simulink model "Gr3_Ex1_3linkedRobot_old"  (R2024b)
settings: Solver=VariableStepAuto  StartTime=0.0  StopTime=10.0  RelTol=1e-3
settings Model: Creator=UX434  LastModifiedBy=UX434

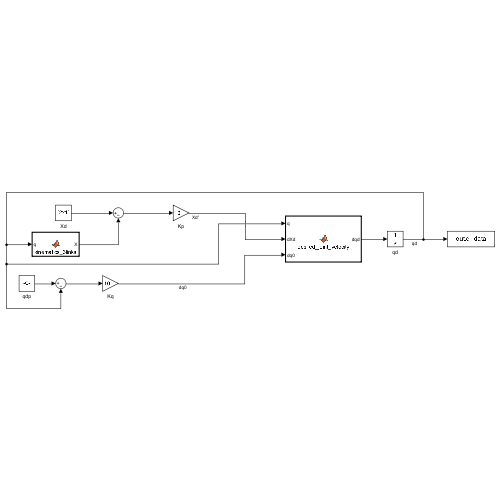
[thumbnail: Simulink's stored preview of the top-level diagram]
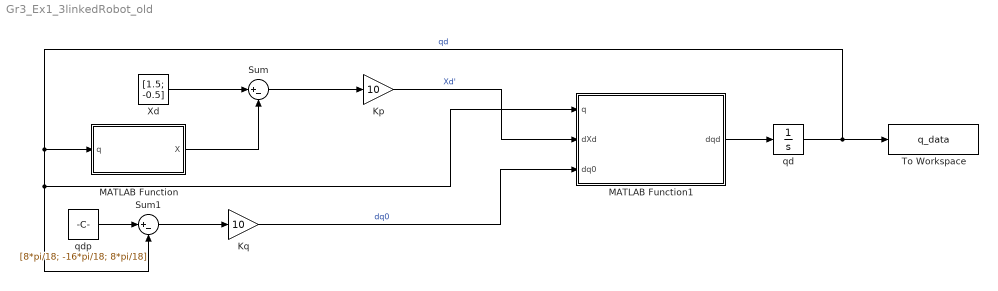
== system Gr3_Ex1_3linkedRobot_old ==
  Kp : Gain  Gain=10
  Kq : Gain  Gain=10
  MATLAB Function : MATLAB Function  TreatAsAtomicUnit=on
  MATLAB Function1 : MATLAB Function  TreatAsAtomicUnit=on
  Sum : Sum  Inputs=|+-
  Sum1 : Sum  Inputs=|+-
  To Workspace : ToWorkspace  VariableName=q_data  SampleTime=-1
  Xd : Constant  Value=[1.5; -0.5]
  qd : Integrator  InitialCondition=[pi/12; pi/3; pi/3]
  qdp : Constant  Value=[8*pi/18; -16*pi/18; 8*pi/18]
  wires:
  qd/1 -> To Workspace/1, MATLAB Function1/1(q), Sum1/2, MATLAB Function/1(q)  "qd"
  MATLAB Function/1(X) -> Sum/2
  Sum/1 -> Kp/1
  Kp/1 -> MATLAB Function1/2(dXd)  "Xd'"
  qdp/1 -> Sum1/1
  Sum1/1 -> Kq/1
  Kq/1 -> MATLAB Function1/3(dq0)  "dq0"
  MATLAB Function1/1(dqd) -> qd/1
  Xd/1 -> Sum/1

== matlab function Gr3_Ex1_3linkedRobot_old/MATLAB Function ==
  data: q input; X output
function X = kinematics_3links(q)
    l1 = 1;  l2 = 1;  l3 = 0.3;
    s1 = sin(q(1));  s12 = sin(q(1)+q(2));  s123 = sin(q(1)+q(2)+q(3));
    c1 = cos(q(1));  c12 = cos(q(1)+q(2));  c123 = cos(q(1)+q(2)+q(3));
    X = [l1*c1 + l2*c12 + l3*c123;
         l1*s1 + l2*s12 + l3*s123];
end

== matlab function Gr3_Ex1_3linkedRobot_old/MATLAB Function1 ==
  data: q input; dqd output; dXd input; dq0 input
function dqd = desired_joint_velocity(q, dXd, dq0)
    l1 = 1;  l2 = 1;  l3 = 0.3;
    s1 = sin(q(1));  s12 = sin(q(1)+q(2));  s123 = sin(q(1)+q(2)+q(3));
    c1 = cos(q(1));  c12 = cos(q(1)+q(2));  c123 = cos(q(1)+q(2)+q(3));

    % Jacobian (2x3)
    J = [-l1*s1-l2*s12-l3*s123, -l2*s12-l3*s123, -l3*s123;
          l1*c1+l2*c12+l3*c123,  l2*c12+l3*c123,  l3*c123];

    % Pseudoinverse J# = J'*inv(J*J')
    Jp = J' / (J*J');

    % dqd = J#*dXd + (I - J#*J)*dq0
    dqd = Jp*dXd + (eye(3) - Jp*J)*dq0;
end
